simulink model "sm_car"  (R2025a)
settings: Solver=ode23t  StartTime=0.0  StopTime=400  MaxStep=0.4  RelTol=1e-3  AbsTol=1e-3  EnableMultiTasking=on
PreLoadFcn:
  | % Due to usability issue in Repeating Sequence block
  | warning('off','Simulink:Masking:Invalid');
  | 
  | % Eliminate unnecessary warnings in inactive variants
  | % Warnings generated only if you click through inactive variant
  | warning('off','MATLAB:nonExistentField');
  | warning('off','Simulink:Parameters:BlkParamUndefined');
PostLoadFcn:
  | set_param([bdroot '/Vehicle'],'popup_trailer','Off')
  | warning('off','sm:sli:setup:compile:LocalSolverNotSupported')
  | %sm_car_config_maneuver(bdroot,'WOT Braking');
  | sm_car_config_vehicle(bdroot,'false');
  | sm_car_config_logging(bdroot);
InitFcn:
  | sm_car_config_camera;
  | Vehicle = sm_car_vehcfg_checkConfig(Vehicle);
  | sm_car_check_tire_model(bdroot);
StartFcn:
  | tic;
StopFcn:
  | Elapsed_Sim_Time = toc;
  | % disp(['Elapsed Sim Time = ' num2str(Elapsed_Sim_Time)]);
undefined symbols (not defined in the file): Axle1D, AxleIn, Camera, Control, Driver, Free, Init, Maneuver, Pedal, RaceFix, RaceSpin, Scene, ShaftL1, ShaftL2, ShaftR1, ShaftR2, Soft, Stiff, Visual, X, xy_data_car_side, Y, Z
libraries: sm_lib x1546, nesl_utility x528, fl_lib x480, SimscapeFluids_lib x61, sdl_lib x49, simulink x29, ee_lib x7, simulink_extras x6, Linkage_Systems x4, Tire_1x2x x4, AntiRollBar_Systems x2, Linkage_Decoupled x2
(part 10 of 79)

== system sm_car/Vehicle/Vehicle/Chassis/Aero/Subsystem ==
  RdBus : Inport
  Actuator dynamics : Subsystem  mask(First-order lag supporting vector signals){b=0.5, x_initial=0}
      mask prompts: b "Filter time constant"; x_initial "Initial output"
      mask help: Models a lag of the form 1/(b*s+1) where s is the Laplace operator.
  Bus Selector : BusSelector  OutputSignals=fx,fy,fz
  Mux : Mux  Inputs=3
  Simulink-PS Converter : nesl_utility/Simulink-PS Converter  PhysicalDomain=network_engine_domain  SubClassName=ps_input  LeftPortType=input  RightPortType=output  PseudoPeriodic=off  Frequencies=[]  NoiseDistribution=none  NoiseParameters=[]  Unit=1  AffineConversion=off  FilteringAndDerivatives=provide  SimscapeFilterOrder=1  InputFilterTimeConstant=0.001  UdotUserProvided=0
  fWind : PMIOPort  Side=Right
  wires:
  Actuator dynamics/1(Out) -> Simulink-PS Converter/1
  RdBus/1 -> Bus Selector/1
  Bus Selector/3 -> Mux/3  "<fz>"
  Bus Selector/2 -> Mux/2  "<fy>"
  Bus Selector/1 -> Mux/1  "<fx>"
  Mux/1 -> Actuator dynamics/1(In)
  connections:
  Simulink-PS Converter/RConn1 -- fWind/RConn1

== system sm_car/Vehicle/Vehicle/Chassis/Body/Body Geometry ==
  CAD FSAE Achilles : Subsystem  VariantControl=CAD_FSAE_Achilles  mask(FSAE Body Geometry){body_offset=BodyGeometry.sOffset.Value, body_orient=BodyGeometry.aOffset.Value, body_clr=BodyGeometry.Color.Value, body_opc=BodyGeometry.Opacity.Value, aero_clr=BodyGeometry.AeroColor.Value, aero_opc=BodyGeometry.AeroOpacity.Value, extr_data_emblem_aero=Visual.PaceCar.emblem.data*0.3, extr_data_emblem_hood=Visual.PaceCar.emblem.data*0.3, clr_emblem_aero=Visual.clr.orange, clr_emblem_hood=Visual.clr.orange, opc_emblem_aero=Visual.emblem.opc, opc_emblem_hood=Visual.emblem.opc}
      mask prompts: body_offset "Body Offset [x y z] (m)"; body_orient "Body Orientation [R P Y] (rad)"; body_clr "Body Color [R G B] (0-1)"; body_opc "Body Opacity (0-1)"; aero_clr "Aero Color [R G B] (0-1)"; aero_opc "Aero Opacity (0-1)"; extr_data_emblem_aero "Emblem Data Aero [xy] (m)"; extr_data_emblem_hood "Emblem Data Hood [xy] (m)"; clr_emblem_aero "Emblem Color Aero [R G B] (0-1)"; clr_emblem_hood "Emblem Color Hood [R G B] (0-1)"; opc_emblem_aero "Emblem Opacity Aero (0-1)"; opc_emblem_hood "Emblem Opacity Hood (0-1)"
      mask help: CAD geometry of Formula Student Vehicle.
      mask TypeOptions extr_data_emblem_aero:
      | Aero/Ornament
      | Left/ExtrusionCrossSection | Aero/Ornament
      | Right/ExtrusionCrossSection
      mask TypeOptions extr_data_emblem_hood:
      | Body/Ornament
      | Hood/ExtrusionCrossSection
      mask TypeOptions clr_emblem_aero:
      | Aero/Ornament
      | Left/GraphicDiffuseColor | Aero/Ornament
      | Right/GraphicDiffuseColor
      mask TypeOptions clr_emblem_hood:
      | Body/Ornament
      | Hood/GraphicDiffuseColor
      mask TypeOptions opc_emblem_aero:
      | Aero/Ornament
      | Left/GraphicOpacity | Aero/Ornament
      | Right/GraphicOpacity
      mask TypeOptions opc_emblem_hood:
      | Body/Ornament
      | Hood/GraphicOpacity
      mask DialogControl cont_emblem Prompt: Emblem
      mask Display: image('sm_car_bodygeometry_cad_fsae_achilles.png');
  FA : PMIOPort  Side=Right
  P : PMIOPort  Port=2  Side=Left

== system sm_car/Vehicle/Vehicle/Chassis/Body/Body Load ==
  None : Subsystem  VariantControl=None
  " FA" : PMIOPort  Side=Left

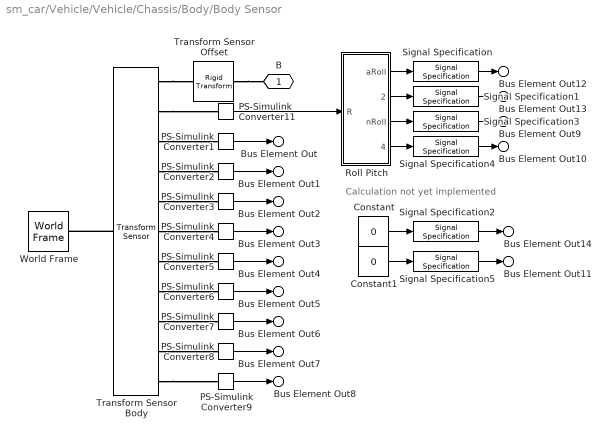
== system sm_car/Vehicle/Vehicle/Chassis/Body/Body Sensor ==
  note: Calculation not yet implemented
  Constant : Constant  Value=0
  Constant1 : Constant  Value=0
  PS-Simulink Converter1 : nesl_utility/PS-Simulink Converter  PhysicalDomain=network_engine_domain  SubClassName=ps_output  LeftPortType=input  RightPortType=output  PseudoPeriodic=off  Frequencies=[]  VectorFormat=1-D array  Unit=m  AffineConversion=off
  PS-Simulink Converter11 : nesl_utility/PS-Simulink Converter  PhysicalDomain=network_engine_domain  SubClassName=ps_output  LeftPortType=input  RightPortType=output  PseudoPeriodic=off  Frequencies=[]  VectorFormat=1-D array  Unit=1  AffineConversion=off
  PS-Simulink Converter2 : nesl_utility/PS-Simulink Converter  PhysicalDomain=network_engine_domain  SubClassName=ps_output  LeftPortType=input  RightPortType=output  PseudoPeriodic=off  Frequencies=[]  VectorFormat=1-D array  Unit=m  AffineConversion=off
  PS-Simulink Converter3 : nesl_utility/PS-Simulink Converter  PhysicalDomain=network_engine_domain  SubClassName=ps_output  LeftPortType=input  RightPortType=output  PseudoPeriodic=off  Frequencies=[]  VectorFormat=1-D array  Unit=m  AffineConversion=off
  PS-Simulink Converter4 : nesl_utility/PS-Simulink Converter  PhysicalDomain=network_engine_domain  SubClassName=ps_output  LeftPortType=input  RightPortType=output  PseudoPeriodic=off  Frequencies=[]  VectorFormat=1-D array  Unit=m/s  AffineConversion=off
  PS-Simulink Converter5 : nesl_utility/PS-Simulink Converter  PhysicalDomain=network_engine_domain  SubClassName=ps_output  LeftPortType=input  RightPortType=output  PseudoPeriodic=off  Frequencies=[]  VectorFormat=1-D array  Unit=m/s  AffineConversion=off
  PS-Simulink Converter6 : nesl_utility/PS-Simulink Converter  PhysicalDomain=network_engine_domain  SubClassName=ps_output  LeftPortType=input  RightPortType=output  PseudoPeriodic=off  Frequencies=[]  VectorFormat=1-D array  Unit=m/s  AffineConversion=off
  PS-Simulink Converter7 : nesl_utility/PS-Simulink Converter  PhysicalDomain=network_engine_domain  SubClassName=ps_output  LeftPortType=input  RightPortType=output  PseudoPeriodic=off  Frequencies=[]  VectorFormat=1-D array  Unit=m/s^2  AffineConversion=off
  PS-Simulink Converter8 : nesl_utility/PS-Simulink Converter  PhysicalDomain=network_engine_domain  SubClassName=ps_output  LeftPortType=input  RightPortType=output  PseudoPeriodic=off  Frequencies=[]  VectorFormat=1-D array  Unit=m/s^2  AffineConversion=off
  PS-Simulink Converter9 : nesl_utility/PS-Simulink Converter  PhysicalDomain=network_engine_domain  SubClassName=ps_output  LeftPortType=input  RightPortType=output  PseudoPeriodic=off  Frequencies=[]  VectorFormat=1-D array  Unit=m/s^2  AffineConversion=off
  Roll Pitch : Subsystem
  Signal Specification : SignalSpecification  Unit=rad
  Signal Specification1 : SignalSpecification  Unit=rad
  Signal Specification2 : SignalSpecification  Unit=rad
  Signal Specification3 : SignalSpecification  Unit=rad/s
  Signal Specification4 : SignalSpecification  Unit=rad/s
  Signal Specification5 : SignalSpecification  Unit=rad/s
  Transform Sensor Offset : sm_lib/Frames and Transforms/Rigid Transform  RotationMethod=None  FollAlignAxisA=+X  BaseAlignAxisA=+Y  FollAlignAxisB=+Y  BaseAlignAxisB=+Z  RotationStandardAxis=+Z  RotationAngle=0.0  RotationAngleUnits=deg  RotationArbitraryAxis=[0 0 1]  RotationSequenceAxes=FollowerAxes  RotationSequence=XYX  RotationSequenceAngles=[0 0 0]  RotationSequenceAnglesUnits=deg  RotationMatrix=[1 0 0; 0 1 0; 0 0 1]  Quaternion=[1 0 0 0]  TranslationMethod=Cartesian  TranslationCartesianOffset=offset_body_sensor  TranslationCartesianOffsetUnits=m  TranslationStandardAxis=+Z  TranslationStandardOffset=0  TranslationStandardOffsetUnits=m  TranslationROffset=0  TranslationROffsetUnits=m  TranslationThetaOffset=0  TranslationThetaOffsetUnits=deg  TranslationZOffset=0  TranslationZOffsetUnits=m
  Transform Sensor Body : sm_lib/Frames and Transforms/Transform Sensor  MeasurementFrame=NonRotatingFollower  RotationSequence=XYX  SenseAngle=off  SenseAxis=off  SenseQ=off  SenseR=on  SenseRotationSequence=off  SenseOmegaX=off  SenseOmegaY=off  SenseOmegaZ=off  SenseOmega=off  SenseQDot=off  SenseRDot=off  SenseRotationSequenceDot=off  SenseAlphaX=off  SenseAlphaY=off  SenseAlphaZ=off  SenseAlpha=off  SenseQDDot=off  SenseRDDot=off  SenseX=on  SenseY=on  SenseZ=on  SenseXYZ=off  SenseRad=off  SenseAzim=off  SenseDist=off  SenseInc=off  SenseXDot=on  SenseYDot=on  SenseZDot=on  SenseXYZDot=off  SenseRadDot=off  SenseAzimDot=off  SenseDistDot=off  SenseIncDot=off  SenseXDDot=on  SenseYDDot=on  SenseZDDot=on  SenseXYZDDot=off  SenseRadDDot=off  SenseAzimDDot=off  SenseDistDDot=off  SenseIncDDot=off
  World Frame : sm_lib/Frames and Transforms/World Frame
  B : PMIOPort  Side=Left
  Bus Element Out : Outport  VectorParamsAs1DForOutWhenUnconnected=off  PortName=Body  Element=x
  Bus Element Out1 : Outport  VectorParamsAs1DForOutWhenUnconnected=off  PortName=Body  Element=y
  Bus Element Out2 : Outport  VectorParamsAs1DForOutWhenUnconnected=off  PortName=Body  Element=z
  Bus Element Out3 : Outport  VectorParamsAs1DForOutWhenUnconnected=off  PortName=Body  Element=vx
  Bus Element Out4 : Outport  VectorParamsAs1DForOutWhenUnconnected=off  PortName=Body  Element=vy
  Bus Element Out5 : Outport  VectorParamsAs1DForOutWhenUnconnected=off  PortName=Body  Element=vz
  Bus Element Out6 : Outport  VectorParamsAs1DForOutWhenUnconnected=off  PortName=Body  Element=gx
  Bus Element Out7 : Outport  VectorParamsAs1DForOutWhenUnconnected=off  PortName=Body  Element=gy
  Bus Element Out8 : Outport  VectorParamsAs1DForOutWhenUnconnected=off  PortName=Body  Element=gz
  Bus Element Out9 : Outport  VectorParamsAs1DForOutWhenUnconnected=off  PortName=Body  Element=nRoll
  Bus Element Out10 : Outport  VectorParamsAs1DForOutWhenUnconnected=off  PortName=Body  Element=nPitch
  Bus Element Out11 : Outport  VectorParamsAs1DForOutWhenUnconnected=off  PortName=Body  Element=nYaw
  Bus Element Out12 : Outport  VectorParamsAs1DForOutWhenUnconnected=off  PortName=Body  Element=aRoll
  Bus Element Out13 : Outport  VectorParamsAs1DForOutWhenUnconnected=off  PortName=Body  Element=aPitch
  Bus Element Out14 : Outport  VectorParamsAs1DForOutWhenUnconnected=off  PortName=Body  Element=aYaw
  wires:
  PS-Simulink Converter9/1 -> Bus Element Out8/1
  PS-Simulink Converter11/1 -> Roll Pitch/1(R)
  PS-Simulink Converter6/1 -> Bus Element Out5/1
  PS-Simulink Converter7/1 -> Bus Element Out6/1
  PS-Simulink Converter2/1 -> Bus Element Out1/1
  PS-Simulink Converter8/1 -> Bus Element Out7/1
  PS-Simulink Converter5/1 -> Bus Element Out4/1
  PS-Simulink Converter3/1 -> Bus Element Out2/1
  PS-Simulink Converter1/1 -> Bus Element Out/1
  PS-Simulink Converter4/1 -> Bus Element Out3/1
  Signal Specification/1 -> Bus Element Out12/1
  Signal Specification1/1 -> Bus Element Out13/1
  Signal Specification2/1 -> Bus Element Out14/1
  Signal Specification3/1 -> Bus Element Out9/1
  Signal Specification4/1 -> Bus Element Out10/1
  Signal Specification5/1 -> Bus Element Out11/1
  Constant/1 -> Signal Specification2/1
  Constant1/1 -> Signal Specification5/1
  Roll Pitch/3(nRoll) -> Signal Specification3/1
  Roll Pitch/4(nPitch) -> Signal Specification4/1
  Roll Pitch/2(aPitch) -> Signal Specification1/1
  Roll Pitch/1(aRoll) -> Signal Specification/1
  connections:
  Transform Sensor Body/RConn5 -- PS-Simulink Converter3/LConn1
  Transform Sensor Body/RConn4 -- PS-Simulink Converter2/LConn1
  Transform Sensor Body/RConn11 -- PS-Simulink Converter9/LConn1
  Transform Sensor Body/RConn2 -- PS-Simulink Converter11/LConn1
  Transform Sensor Body/RConn7 -- PS-Simulink Converter5/LConn1
  Transform Sensor Body/RConn3 -- PS-Simulink Converter1/LConn1
  Transform Sensor Body/LConn1 -- World Frame/RConn1
  Transform Sensor Offset/LConn1 -- B/RConn1
  Transform Sensor Body/RConn10 -- PS-Simulink Converter8/LConn1
  Transform Sensor Body/RConn9 -- PS-Simulink Converter7/LConn1
  Transform Sensor Body/RConn8 -- PS-Simulink Converter6/LConn1
  Transform Sensor Body/RConn6 -- PS-Simulink Converter4/LConn1
  Transform Sensor Body/RConn1 -- Transform Sensor Offset/RConn1

== system sm_car/Vehicle/Vehicle/Chassis/Body/Passenger FL ==
  None : Subsystem  VariantControl=None
      mask Display: disp(' ')
  P : PMIOPort  Side=Left
  m : Outport  VectorParamsAs1DForOutWhenUnconnected=off

== system sm_car/Vehicle/Vehicle/Chassis/Body/Passenger FR ==
  None : Subsystem  VariantControl=None
      mask Display: disp(' ')
  P : PMIOPort  Side=Left
  m : Outport  VectorParamsAs1DForOutWhenUnconnected=off

== system sm_car/Vehicle/Vehicle/Chassis/Body/Passenger RL ==
  None : Subsystem  VariantControl=None
      mask Display: disp(' ')
  P : PMIOPort  Side=Left
  m : Outport  VectorParamsAs1DForOutWhenUnconnected=off

== system sm_car/Vehicle/Vehicle/Chassis/Body/Passenger RR ==
  None : Subsystem  VariantControl=None
      mask Display: disp(' ')
  P : PMIOPort  Side=Left
  m : Outport  VectorParamsAs1DForOutWhenUnconnected=off

== system sm_car/Vehicle/Vehicle/Chassis/Damper/Decoupled ==
  In Bus Element1 : Inport  PortName=Ctrl  Element=L1
  In Bus Element : Inport  PortName=Ctrl  Element=R1
  In Bus Element2 : Inport  PortName=Ctrl  Element=L2
  In Bus Element3 : Inport  PortName=Ctrl  Element=R2
  Damper A1 Heave : Subsystem  Variant=on  VariantControlMode=label  VariantControl=Variant1  LabelModeActiveChoice=Linear  mask(Variants for Damper){Damper=Damper.Axle1.Heave, VariantLabel=Damper.Axle1.Heave.class.Value}
      mask prompts: Damper "Damper Parameters"; VariantLabel "Variant Label"
      mask help: Select option and provide parameters for damper. Option is chosen by string provided in Variant Label. The parameters for the selected option is contained in Damper data structure.
      mask init:
      | curblk = gcb;
      | 
      | % Set variant for this block 
      | set_param(curblk,'LabelModeActiveChoice',VariantLabel);
      settings: AttributesFormatString=%<ActiveVariant>
      mask Display: disp(' ')
  Damper A1 Roll : Subsystem  Variant=on  VariantControlMode=label  VariantControl=Variant1  LabelModeActiveChoice=Linear  mask(Variants for Damper){Damper=Damper.Axle1.Roll, VariantLabel=Damper.Axle1.Roll.class.Value}
      mask prompts: Damper "Damper Parameters"; VariantLabel "Variant Label"
      mask help: Select option and provide parameters for damper. Option is chosen by string provided in Variant Label. The parameters for the selected option is contained in Damper data structure.
      mask init:
      | curblk = gcb;
      | 
      | % Set variant for this block 
      | set_param(curblk,'LabelModeActiveChoice',VariantLabel);
      settings: AttributesFormatString=%<ActiveVariant>
      mask Display: disp(' ')
  Damper A2 Heave : Subsystem  Variant=on  VariantControlMode=label  VariantControl=Variant1  LabelModeActiveChoice=Linear  mask(Variants for Damper){Damper=Damper.Axle2.Heave, VariantLabel=Damper.Axle2.Heave.class.Value}
      mask prompts: Damper "Damper Parameters"; VariantLabel "Variant Label"
      mask help: Select option and provide parameters for damper. Option is chosen by string provided in Variant Label. The parameters for the selected option is contained in Damper data structure.
      mask init:
      | curblk = gcb;
      | 
      | % Set variant for this block 
      | set_param(curblk,'LabelModeActiveChoice',VariantLabel);
      settings: AttributesFormatString=%<ActiveVariant>
      mask Display: disp(' ')
  Damper A2 Roll : Subsystem  Variant=on  VariantControlMode=label  VariantControl=Variant1  LabelModeActiveChoice=Linear  mask(Variants for Damper){Damper=Damper.Axle2.Roll, VariantLabel=Damper.Axle2.Roll.class.Value}
      mask prompts: Damper "Damper Parameters"; VariantLabel "Variant Label"
      mask help: Select option and provide parameters for damper. Option is chosen by string provided in Variant Label. The parameters for the selected option is contained in Damper data structure.
      mask init:
      | curblk = gcb;
      | 
      | % Set variant for this block 
      | set_param(curblk,'LabelModeActiveChoice',VariantLabel);
      settings: AttributesFormatString=%<ActiveVariant>
      mask Display: disp(' ')
  MTRef L1 : fl_lib/Mechanical/Translational Elements/Mechanical Translational Reference
  MTRef L2 : fl_lib/Mechanical/Translational Elements/Mechanical Translational Reference
  MTRef R1 : fl_lib/Mechanical/Translational Elements/Mechanical Translational Reference
  MTRef R2 : fl_lib/Mechanical/Translational Elements/Mechanical Translational Reference
  L1 : PMIOPort  Side=Left
  R1 : PMIOPort  Port=2  Side=Right
  L2 : PMIOPort  Port=3  Side=Left
  R2 : PMIOPort  Port=4  Side=Right
  Out Bus Element : Outport  VectorParamsAs1DForOutWhenUnconnected=off  PortName=meas  Element=L1
  Out Bus Element1 : Outport  VectorParamsAs1DForOutWhenUnconnected=off  PortName=meas  Element=R1
  Out Bus Element2 : Outport  VectorParamsAs1DForOutWhenUnconnected=off  PortName=meas  Element=L2
  Out Bus Element3 : Outport  VectorParamsAs1DForOutWhenUnconnected=off  PortName=meas  Element=R2
  wires:
  In Bus Element/1 -> Damper A1 Roll/1("Ctrl ")
  In Bus Element1/1 -> Damper A1 Heave/1("Ctrl ")
  Damper A1 Heave/1(" meas") -> Out Bus Element/1
  Damper A1 Roll/1(" meas") -> Out Bus Element1/1
  In Bus Element3/1 -> Damper A2 Roll/1("Ctrl ")
  In Bus Element2/1 -> Damper A2 Heave/1("Ctrl ")
  Damper A2 Heave/1(" meas") -> Out Bus Element2/1
  Damper A2 Roll/1(" meas") -> Out Bus Element3/1
  connections:
  Damper A1 Roll/LConn1 -- R1/RConn1
  Damper A1 Roll/RConn1 -- MTRef R1/LConn1
  Damper A2 Roll/LConn1 -- R2/RConn1
  Damper A2 Roll/RConn1 -- MTRef R2/LConn1
  Damper A2 Heave/LConn1 -- L2/RConn1
  Damper A2 Heave/RConn1 -- MTRef L2/LConn1
  Damper A1 Heave/LConn1 -- L1/RConn1
  Damper A1 Heave/RConn1 -- MTRef L1/LConn1

== system sm_car/Vehicle/Vehicle/Chassis/Damper/Independent ==
  In Bus Element1 : Inport  PortName=Ctrl  Element=L1
  In Bus Element : Inport  PortName=Ctrl  Element=R1
  In Bus Element2 : Inport  PortName=Ctrl  Element=L2
  In Bus Element3 : Inport  PortName=Ctrl  Element=R2
  Damper L1 : Subsystem  Variant=on  VariantControlMode=label  VariantControl=Variant1  LabelModeActiveChoice=Linear  mask(Variants for Damper){Damper=Damper.Axle1, VariantLabel=Damper.Axle1.class.Value}
      mask prompts: Damper "Damper Parameters"; VariantLabel "Variant Label"
      mask help: Select option and provide parameters for damper. Option is chosen by string provided in Variant Label. The parameters for the selected option is contained in Damper data structure.
      mask init:
      | curblk = gcb;
      | 
      | % Set variant for this block 
      | set_param(curblk,'LabelModeActiveChoice',VariantLabel);
      settings: AttributesFormatString=%<ActiveVariant>
      mask Display: disp(' ')
  Damper L2 : Subsystem  Variant=on  VariantControlMode=label  VariantControl=Variant1  LabelModeActiveChoice=Linear  mask(Variants for Damper){Damper=Damper.Axle2, VariantLabel=Damper.Axle2.class.Value}
      mask prompts: Damper "Damper Parameters"; VariantLabel "Variant Label"
      mask help: Select option and provide parameters for damper. Option is chosen by string provided in Variant Label. The parameters for the selected option is contained in Damper data structure.
      mask init:
      | curblk = gcb;
      | 
      | % Set variant for this block 
      | set_param(curblk,'LabelModeActiveChoice',VariantLabel);
      settings: AttributesFormatString=%<ActiveVariant>
      mask Display: disp(' ')
  Damper R1 : Subsystem  Variant=on  VariantControlMode=label  VariantControl=Variant1  LabelModeActiveChoice=Linear  mask(Variants for Damper){Damper=Damper.Axle1, VariantLabel=Damper.Axle1.class.Value}
      mask prompts: Damper "Damper Parameters"; VariantLabel "Variant Label"
      mask help: Select option and provide parameters for damper. Option is chosen by string provided in Variant Label. The parameters for the selected option is contained in Damper data structure.
      mask init:
      | curblk = gcb;
      | 
      | % Set variant for this block 
      | set_param(curblk,'LabelModeActiveChoice',VariantLabel);
      settings: AttributesFormatString=%<ActiveVariant>
      mask Display: disp(' ')
  Damper R2 : Subsystem  Variant=on  VariantControlMode=label  VariantControl=Variant1  LabelModeActiveChoice=Linear  mask(Variants for Damper){Damper=Damper.Axle2, VariantLabel=Damper.Axle2.class.Value}
      mask prompts: Damper "Damper Parameters"; VariantLabel "Variant Label"
      mask help: Select option and provide parameters for damper. Option is chosen by string provided in Variant Label. The parameters for the selected option is contained in Damper data structure.
      mask init:
      | curblk = gcb;
      | 
      | % Set variant for this block 
      | set_param(curblk,'LabelModeActiveChoice',VariantLabel);
      settings: AttributesFormatString=%<ActiveVariant>
      mask Display: disp(' ')
  MTRef L1 : fl_lib/Mechanical/Translational Elements/Mechanical Translational Reference
  MTRef L2 : fl_lib/Mechanical/Translational Elements/Mechanical Translational Reference
  MTRef R1 : fl_lib/Mechanical/Translational Elements/Mechanical Translational Reference
  MTRef R2 : fl_lib/Mechanical/Translational Elements/Mechanical Translational Reference
  L1 : PMIOPort  Side=Left
  R1 : PMIOPort  Port=2  Side=Right
  L2 : PMIOPort  Port=3  Side=Left
  R2 : PMIOPort  Port=4  Side=Right
  Out Bus Element : Outport  VectorParamsAs1DForOutWhenUnconnected=off  PortName=meas  Element=L1
  Out Bus Element1 : Outport  VectorParamsAs1DForOutWhenUnconnected=off  PortName=meas  Element=R1
  Out Bus Element2 : Outport  VectorParamsAs1DForOutWhenUnconnected=off  PortName=meas  Element=L2
  Out Bus Element3 : Outport  VectorParamsAs1DForOutWhenUnconnected=off  PortName=meas  Element=R2
  wires:
  In Bus Element/1 -> Damper R1/1("Ctrl ")
  In Bus Element1/1 -> Damper L1/1("Ctrl ")
  Damper L1/1(" meas") -> Out Bus Element/1
  Damper R1/1(" meas") -> Out Bus Element1/1
  In Bus Element3/1 -> Damper R2/1("Ctrl ")
  In Bus Element2/1 -> Damper L2/1("Ctrl ")
  Damper L2/1(" meas") -> Out Bus Element2/1
  Damper R2/1(" meas") -> Out Bus Element3/1
  connections:
  Damper R1/LConn1 -- R1/RConn1
  Damper R1/RConn1 -- MTRef R1/LConn1
  Damper R2/LConn1 -- R2/RConn1
  Damper R2/RConn1 -- MTRef R2/LConn1
  Damper L2/LConn1 -- L2/RConn1
  Damper L2/RConn1 -- MTRef L2/LConn1
  Damper L1/LConn1 -- L1/RConn1
  Damper L1/RConn1 -- MTRef L1/LConn1

== system sm_car/Vehicle/Vehicle/Chassis/Spring/Decoupled ==
  In Bus Element1 : Inport  PortName=Ctrl  Element=L1
  In Bus Element2 : Inport  PortName=Ctrl  Element=R1
  In Bus Element3 : Inport  PortName=Ctrl  Element=L2
  In Bus Element4 : Inport  PortName=Ctrl  Element=R2
  MTRef Heave A1 : fl_lib/Mechanical/Translational Elements/Mechanical Translational Reference
  MTRef Heave A2 : fl_lib/Mechanical/Translational Elements/Mechanical Translational Reference
  MTRef Roll A1 : fl_lib/Mechanical/Translational Elements/Mechanical Translational Reference
  MTRef Roll A2 : fl_lib/Mechanical/Translational Elements/Mechanical Translational Reference
  Spring A1 Heave : Subsystem  Variant=on  VariantControlMode=label  VariantControl=Variant1  LabelModeActiveChoice=Linear  mask(Variants for Spring){Spring=Spring.Axle1.Heave, VariantLabel=Spring.Axle1.Heave.class.Value}
      mask prompts: Spring "Spring Parameters"; VariantLabel "Variant Label"
      mask help: Select option and provide parameters for spring. Option is chosen by string provided in Variant Label. The parameters for the selected option is contained in Spring data structure.
      mask init:
      | curblk = gcb;
      | 
      | % Set variant for this block 
      | set_param(curblk,'LabelModeActiveChoice',VariantLabel);
      settings: AttributesFormatString=%<ActiveVariant>
      mask Display: disp(' ')
  Spring A1 Roll : Subsystem  Variant=on  VariantControlMode=label  VariantControl=Variant1  LabelModeActiveChoice=Linear  mask(Variants for Spring){Spring=Spring.Axle1.Roll, VariantLabel=Spring.Axle1.Roll.class.Value}
      mask prompts: Spring "Spring Parameters"; VariantLabel "Variant Label"
      mask help: Select option and provide parameters for spring. Option is chosen by string provided in Variant Label. The parameters for the selected option is contained in Spring data structure.
      mask init:
      | curblk = gcb;
      | 
      | % Set variant for this block 
      | set_param(curblk,'LabelModeActiveChoice',VariantLabel);
      settings: AttributesFormatString=%<ActiveVariant>
      mask Display: disp(' ')
  Spring A2 Heave : Subsystem  Variant=on  VariantControlMode=label  VariantControl=Variant1  LabelModeActiveChoice=Linear  mask(Variants for Spring){Spring=Spring.Axle2.Heave, VariantLabel=Spring.Axle2.Heave.class.Value}
      mask prompts: Spring "Spring Parameters"; VariantLabel "Variant Label"
      mask help: Select option and provide parameters for spring. Option is chosen by string provided in Variant Label. The parameters for the selected option is contained in Spring data structure.
      mask init:
      | curblk = gcb;
      | 
      | % Set variant for this block 
      | set_param(curblk,'LabelModeActiveChoice',VariantLabel);
      settings: AttributesFormatString=%<ActiveVariant>
      mask Display: disp(' ')
  Spring A2 Roll : Subsystem  Variant=on  VariantControlMode=label  VariantControl=Variant1  LabelModeActiveChoice=Linear  mask(Variants for Spring){Spring=Spring.Axle2.Roll, VariantLabel=Spring.Axle2.Roll.class.Value}
      mask prompts: Spring "Spring Parameters"; VariantLabel "Variant Label"
      mask help: Select option and provide parameters for spring. Option is chosen by string provided in Variant Label. The parameters for the selected option is contained in Spring data structure.
      mask init:
      | curblk = gcb;
      | 
      | % Set variant for this block 
      | set_param(curblk,'LabelModeActiveChoice',VariantLabel);
      settings: AttributesFormatString=%<ActiveVariant>
      mask Display: disp(' ')
  L1 : PMIOPort  Side=Left
  R1 : PMIOPort  Port=2  Side=Right
  L2 : PMIOPort  Port=3  Side=Left
  R2 : PMIOPort  Port=4  Side=Right
  Out Bus Element : Outport  VectorParamsAs1DForOutWhenUnconnected=off  PortName=meas  Element=L1
  Out Bus Element1 : Outport  VectorParamsAs1DForOutWhenUnconnected=off  PortName=meas  Element=R1
  Out Bus Element2 : Outport  VectorParamsAs1DForOutWhenUnconnected=off  PortName=meas  Element=L2
  Out Bus Element3 : Outport  VectorParamsAs1DForOutWhenUnconnected=off  PortName=meas  Element=R2
  wires:
  In Bus Element1/1 -> Spring A1 Heave/1("Ctrl ")
  Spring A1 Heave/1(" meas") -> Out Bus Element/1
  In Bus Element2/1 -> Spring A1 Roll/1("Ctrl ")
  Spring A1 Roll/1(" meas") -> Out Bus Element1/1
  In Bus Element3/1 -> Spring A2 Heave/1("Ctrl ")
  Spring A2 Heave/1(" meas") -> Out Bus Element2/1
  In Bus Element4/1 -> Spring A2 Roll/1("Ctrl ")
  Spring A2 Roll/1(" meas") -> Out Bus Element3/1
  connections:
  Spring A1 Roll/LConn1 -- R1/RConn1
  Spring A1 Roll/RConn1 -- MTRef Roll A1/LConn1
  Spring A2 Roll/LConn1 -- R2/RConn1
  Spring A2 Roll/RConn1 -- MTRef Roll A2/LConn1
  Spring A2 Heave/LConn1 -- L2/RConn1
  Spring A2 Heave/RConn1 -- MTRef Heave A2/LConn1
  Spring A1 Heave/LConn1 -- L1/RConn1
  Spring A1 Heave/RConn1 -- MTRef Heave A1/LConn1

== system sm_car/Vehicle/Vehicle/Chassis/Spring/Independent ==
  In Bus Element1 : Inport  PortName=Ctrl  Element=L1
  In Bus Element2 : Inport  PortName=Ctrl  Element=R1
  In Bus Element3 : Inport  PortName=Ctrl  Element=L2
  In Bus Element4 : Inport  PortName=Ctrl  Element=R2
  MTRef L1 : fl_lib/Mechanical/Translational Elements/Mechanical Translational Reference
  MTRef L2 : fl_lib/Mechanical/Translational Elements/Mechanical Translational Reference
  MTRef R1 : fl_lib/Mechanical/Translational Elements/Mechanical Translational Reference
  MTRef R2 : fl_lib/Mechanical/Translational Elements/Mechanical Translational Reference
  Spring L1 : Subsystem  Variant=on  VariantControlMode=label  VariantControl=Variant1  LabelModeActiveChoice=Linear  mask(Variants for Spring){Spring=Spring.Axle1, VariantLabel=Spring.Axle1.class.Value}
      mask prompts: Spring "Spring Parameters"; VariantLabel "Variant Label"
      mask help: Select option and provide parameters for spring. Option is chosen by string provided in Variant Label. The parameters for the selected option is contained in Spring data structure.
      mask init:
      | curblk = gcb;
      | 
      | % Set variant for this block 
      | set_param(curblk,'LabelModeActiveChoice',VariantLabel);
      settings: AttributesFormatString=%<ActiveVariant>
      mask Display: disp(' ')
  Spring L2 : Subsystem  Variant=on  VariantControlMode=label  VariantControl=Variant1  LabelModeActiveChoice=Linear  mask(Variants for Spring){Spring=Spring.Axle2, VariantLabel=Spring.Axle2.class.Value}
      mask prompts: Spring "Spring Parameters"; VariantLabel "Variant Label"
      mask help: Select option and provide parameters for spring. Option is chosen by string provided in Variant Label. The parameters for the selected option is contained in Spring data structure.
      mask init:
      | curblk = gcb;
      | 
      | % Set variant for this block 
      | set_param(curblk,'LabelModeActiveChoice',VariantLabel);
      settings: AttributesFormatString=%<ActiveVariant>
      mask Display: disp(' ')
  Spring R1 : Subsystem  Variant=on  VariantControlMode=label  VariantControl=Variant1  LabelModeActiveChoice=Linear  mask(Variants for Spring){Spring=Spring.Axle1, VariantLabel=Spring.Axle1.class.Value}
      mask prompts: Spring "Spring Parameters"; VariantLabel "Variant Label"
      mask help: Select option and provide parameters for spring. Option is chosen by string provided in Variant Label. The parameters for the selected option is contained in Spring data structure.
      mask init:
      | curblk = gcb;
      | 
      | % Set variant for this block 
      | set_param(curblk,'LabelModeActiveChoice',VariantLabel);
      settings: AttributesFormatString=%<ActiveVariant>
      mask Display: disp(' ')
  Spring R2 : Subsystem  Variant=on  VariantControlMode=label  VariantControl=Variant1  LabelModeActiveChoice=Linear  mask(Variants for Spring){Spring=Spring.Axle2, VariantLabel=Spring.Axle2.class.Value}
      mask prompts: Spring "Spring Parameters"; VariantLabel "Variant Label"
      mask help: Select option and provide parameters for spring. Option is chosen by string provided in Variant Label. The parameters for the selected option is contained in Spring data structure.
      mask init:
      | curblk = gcb;
      | 
      | % Set variant for this block 
      | set_param(curblk,'LabelModeActiveChoice',VariantLabel);
      settings: AttributesFormatString=%<ActiveVariant>
      mask Display: disp(' ')
  L1 : PMIOPort  Side=Left
  R1 : PMIOPort  Port=2  Side=Right
  L2 : PMIOPort  Port=3  Side=Left
  R2 : PMIOPort  Port=4  Side=Right
  Out Bus Element : Outport  VectorParamsAs1DForOutWhenUnconnected=off  PortName=meas  Element=L1
  Out Bus Element1 : Outport  VectorParamsAs1DForOutWhenUnconnected=off  PortName=meas  Element=R1
  Out Bus Element2 : Outport  VectorParamsAs1DForOutWhenUnconnected=off  PortName=meas  Element=L2
  Out Bus Element3 : Outport  VectorParamsAs1DForOutWhenUnconnected=off  PortName=meas  Element=R2
  wires:
  In Bus Element1/1 -> Spring L1/1("Ctrl ")
  Spring L1/1(" meas") -> Out Bus Element/1
  In Bus Element2/1 -> Spring R1/1("Ctrl ")
  Spring R1/1(" meas") -> Out Bus Element1/1
  In Bus Element3/1 -> Spring L2/1("Ctrl ")
  Spring L2/1(" meas") -> Out Bus Element2/1
  In Bus Element4/1 -> Spring R2/1("Ctrl ")
  Spring R2/1(" meas") -> Out Bus Element3/1
  connections:
  Spring R1/LConn1 -- R1/RConn1
  Spring R1/RConn1 -- MTRef R1/LConn1
  Spring R2/LConn1 -- R2/RConn1
  Spring R2/RConn1 -- MTRef R2/LConn1
  Spring L2/LConn1 -- L2/RConn1
  Spring L2/RConn1 -- MTRef L2/LConn1
  Spring L1/LConn1 -- L1/RConn1
  Spring L1/RConn1 -- MTRef L1/LConn1

== system sm_car/Vehicle/Vehicle/Chassis/SuspA1/Linkage ==
  In Bus Element : Inport  PortName=CtrlBus  Element=Steer
  DrvBus : Inport  Port=2
  Anti Roll Bar : AntiRollBar_Systems/Anti Roll Bar  LabelModeActiveChoice=DroplinkRod  AntiRollBar=Susp.AntiRollBar  VariantLabel=Susp.AntiRollBar.class.Value
      settings: AttributesFormatString=%<LabelModeActiveChoice>
  Linkage L : Linkage_Systems/Linkage  VariantControl=Variant1  LabelModeActiveChoice=DoubleWishbone  popup_leftRight=Left  Linkage=Susp.Linkage  InitLinkage=Init  VariantLabel=Susp.Linkage.class.Value
      settings: AttributesFormatString=%<ActiveVariant>
  Linkage R : Linkage_Systems/Linkage  Tag=PublishSubsystem  VariantControl=Variant1  LabelModeActiveChoice=DoubleWishbone  popup_leftRight=Right  Linkage=Susp.Linkage  InitLinkage=Init  VariantLabel=Susp.Linkage.class.Value
      settings: AttributesFormatString=%<ActiveVariant>
  Simscape Bus L : SimscapeBus  HierarchyStrings=RaceSpin;RaceFix;Axle1D;AxleIn
  Simscape Bus L1 : SimscapeBus  HierarchyStrings=RaceSpin;RaceFix;Axle1D;AxleIn
  Steer : Subsystem  Variant=on  VariantControlMode=label  VariantControl=Steer  LabelModeActiveChoice=WheelDrivenRack1UJoint  mask(Steering System with Rack){Steer=Susp.Steer, VariantLabel=Susp.Steer.class.Value}
      mask prompts: Steer "Steer Parameters"; VariantLabel "Variant Label"
      mask help: Models steering system that involves a rack. Optionally include steering wheel. Connection between steering wheel and rack can be mechanical, specified by a lookup table, or a control system as in steer-by-wire. Option is chosen by string provided in Variant Label. The parameters for the selected option are contained in Steer data structure.
      mask init:
      | curblk = gcb;
      | 
      | % Set variant for this block 
      | set_param(curblk,'LabelModeActiveChoice',VariantLabel);
      settings: AttributesFormatString=%<ActiveVariant>
      mask Display: disp(' ');
  Wheel Meas Left : Subsystem  mask(Wheel Measurements){popup_leftRight=Left}
      mask prompts: popup_leftRight "Left/Right"
      mask help: Calculates toe and camber angles based on orientation of wheel spin axis. To estimate steering axis inclination, the same measurements are done along the longitudinal axis (X) of the tire. Set Left/Right so that the sign of the logged toe and camber angles is associated with towards/away from vehicle center.
      mask init:
      | if(popup_leftRight == 1)
      |     rhs_tc = 1;
      | elseif(popup_leftRight == 2)
      |     rhs_tc = -1;
      | end
      mask TypeOptions popup_leftRight: Left | Right
  Wheel Meas Right : Subsystem  mask(Wheel Measurements){popup_leftRight=Right}
      mask prompts: popup_leftRight "Left/Right"
      mask help: Calculates toe and camber angles based on orientation of wheel spin axis. To estimate steering axis inclination, the same measurements are done along the longitudinal axis (X) of the tire. Set Left/Right so that the sign of the logged toe and camber angles is associated with towards/away from vehicle center.
      mask init:
      | if(popup_leftRight == 1)
      |     rhs_tc = 1;
      | elseif(popup_leftRight == 2)
      |     rhs_tc = -1;
      | end
      mask TypeOptions popup_leftRight: Left | Right
  WCL : PMIOPort  Side=Left
  Ref : PMIOPort  Port=2  Side=Right
  WCR : PMIOPort  Port=3  Side=Right
  AxleL : PMIOPort  Port=4  Side=Left
  AxleR : PMIOPort  Port=5  Side=Right
  SprL : PMIOPort  Port=6  Side=Left
  SprR : PMIOPort  Port=7  Side=Right
  DmpL : PMIOPort  Port=8  Side=Left
  DmpR : PMIOPort  Port=9  Side=Right
  Out Bus Element : Outport  VectorParamsAs1DForOutWhenUnconnected=off  PortName=OutBus  Element=Steer
  Out Bus Element1 : Outport  VectorParamsAs1DForOutWhenUnconnected=off  PortName=OutBus  Element=AntiRollBar
  Out Bus Element2 : Outport  VectorParamsAs1DForOutWhenUnconnected=off  PortName=OutBus  Element=WhlL
  Out Bus Element3 : Outport  VectorParamsAs1DForOutWhenUnconnected=off  PortName=OutBus  Element=WhlR
  Out Bus Element4 : Outport  VectorParamsAs1DForOutWhenUnconnected=off  PortName=OutBus  Element=LinkageR
  Out Bus Element5 : Outport  VectorParamsAs1DForOutWhenUnconnected=off  PortName=OutBus  Element=LinkageL
  wires:
  Linkage L/1 -> Out Bus Element5/1
  Linkage R/1 -> Out Bus Element4/1
  DrvBus/1 -> Steer/1(DrvBus)
  Steer/1(" meas") -> Out Bus Element/1
  In Bus Element/1 -> Steer/2(CtrlBus)
  Anti Roll Bar/1 -> Out Bus Element1/1
  Wheel Meas Left/1(meas) -> Out Bus Element2/1
  Wheel Meas Right/1(meas) -> Out Bus Element3/1
  connections:
  Steer/RConn3 -- Linkage R/RConn1
  Ref/RConn1 -- Anti Roll Bar/LConn2 -- Linkage R/RConn2 -- Wheel Meas Right/LConn1 -- Wheel Meas Left/LConn1 -- Steer/RConn2 -- Linkage L/RConn2
  Linkage L/LConn1 -- WCL/RConn1 -- Wheel Meas Left/LConn2
  Linkage R/LConn1 -- WCR/RConn1 -- Wheel Meas Right/LConn2
  Steer/RConn1 -- Linkage L/RConn1
  DmpL/RConn1 -- Linkage L/LConn7
  Simscape Bus L/LConn4 -- Linkage L/LConn5
  Simscape Bus L/LConn1 -- Linkage L/LConn2
  Linkage L/LConn3 -- Simscape Bus L/LConn2
  Linkage L/LConn4 -- Simscape Bus L/LConn3
  AxleL/RConn1 -- Simscape Bus L/RConn1
  DmpR/RConn1 -- Linkage R/LConn7
  SprR/RConn1 -- Linkage R/LConn6
  Simscape Bus L1/LConn1 -- Linkage R/LConn2
  Simscape Bus L1/LConn2 -- Linkage R/LConn3
  Simscape Bus L1/LConn3 -- Linkage R/LConn4
  Simscape Bus L1/RConn1 -- AxleR/RConn1
  SprL/RConn1 -- Linkage L/LConn6
  Simscape Bus L1/LConn4 -- Linkage R/LConn5
  Anti Roll Bar/LConn3 -- Linkage R/LConn8
  Anti Roll Bar/LConn1 -- Linkage L/LConn8
